simulink model "PassVeh14DOF"  (R2026b)
settings: Solver=ode23tb  StopTime=inf  FixedStep=.001  RelTol=1e-1  EnableMultiTasking=on
model workspace (MAT data in the model file):
  AlgnTrqCambCompl = [0 0 0 0]
  AlgnTrqSteerCompl = [0 0 0 0]
  AxlIxx = 62.3745166667
  AxlM = 160
  BumpCamber = [0 0 0 0]
  BumpCaster = [0 0 0 0]
  BumpSteer = [0 0 0 0]
  CambVsSteerAng = [0 0 0 0]
  CastVsSteerAng = [0 0 0 0]
  Cps = 2
  Cz = 5565.2246438
  CzWhlAxl = 11490.971257
  DCT_Param : object (value not decoded)
  Downshift_Speeds = [9.5625 12.9375 16.3125 19.6875 23.0625 26.4375 29.8125 33.1875 36.5625 39.9375 43.3125 46.6875 ... (28 elements, 4x7)]
  F0z = [2886 2907]
  F0zWhlAxl = 2907
  Hmax = 0.25
  Kz = 52451.0065793
  KzWhlAxl = 138031.612078
  LatCambCompl = [0 0 0 0]
  LatSteerCompl = [0 0 0 0]
  LatWhlCtrComplLat = [0 0 0 0]
  LatWhlCtrComplLng = [0  0  0  0; 0  0  0  0]
  LatWhlCtrDisp = [0 0 0 0]
  LngCambCompl = [0  0  0  0; 0  0  0  0]
  LngCastCompl = [0  0  0  0; 0  0  0  0]
  LngSteerCompl = [0  0  0  0; 0  0  0  0]
  LngWhlCtrCompl = [0  0  0  0; 0  0  0  0]
  LngWhlCtrDisp = [0 0 0 0]
  MotRatios = [1 1]
  NCyl = 6
  NrmlWhlFrcOff = [2886 2886 2907 2907]
  NrmlWhlRates = [52.4510065793 52.4510065793 52.4510065793 52.4510065793]
  Pedal_Positions = [0.1 0.4 0.5 0.9]
  Pstd = 101325
  Rair = 287
  RollCamber : object (value not decoded)
  RollCaster : object (value not decoded)
  RollSteer : object (value not decoded)
  RollStiffArb = [0 0]
  RollStiffArbFrnt = 800
  RollStiffNoArb = [0 0]
  RollStiffNoArbFrnt = 0
  RollStiffNoTwstRear = 0
  ShckFrcVsCompRate = [5.5652246438 5.5652246438 5.5652246438 5.5652246438]
  StatCamber = [0 0 0 0]
  StatCaster = [0 0 0 0]
  StatLdWhlR = [0.3 0.3 0.3 0.3]
  StatToe = [0 0 0 0]
  Trans : object (value not decoded)
  Tstd = 293.15
  Upshift_Speeds = [12.9375 16.3125 19.6875 33 26.4375 29.8125 33.1875 52.5 39.9375 43.3125 46.6875 77.25 ... (28 elements, 4x7)]
  VEH : object (value not decoded)
  Vd = 0.00346
  VrtLdTrnsfr = [0 0 0 0]
  WH : Mass (value not decoded)
  dt3D = 0.05
  f_air = [0 0 0 0 0 0 0 0 0 0 0 0 ... (256 elements, 16x16)]
  f_co = [0 0 0 0 0 0 0 0 0 0 0 0 ... (256 elements, 16x16)]
  f_co2 = [0 0 0 0 0 0 0 0 0 0 0 0 ... (256 elements, 16x16)]
  f_eff = [352.135682859 352.135682859 320.724378192 303.655312657 295.930136708 291.240087194 291.240271258 291.240312459 291.240275452 291.240198499 291.240100781 291.240018769 ... (256 elements, 16x16)]
  f_fuel = [0 0 0 0 0 0 0 0 0 0 0 0 ... (256 elements, 16x16)]
  f_hc = [0 0 0 0 0 0 0 0 0 0 0 0 ... (256 elements, 16x16)]
  f_nox = [0 0 0 0 0 0 0 0 0 0 0 0 ... (256 elements, 16x16)]
  f_pm = [0 0 0 0 0 0 0 0 0 0 0 0 ... (256 elements, 16x16)]
  f_susp_axl_bp = [1 2]
  f_susp_dz_bp = [-0.325022776267 -0.315022776267 -0.305022776267 -0.205022776267 -0.105022776267 -0.00502277626717 0.0949772237328 0.194977223733 0.204977223733 0.214977223733]
  f_susp_dzdot_bp = [-3 -0.3 -0.2 -0.1 0 0.1 0.2 0.3 3]
  f_susp_fmz = [-144070.391448 -93629.24037 -75929.1118915 -20630.5828179 -15385.48216 -10140.3815021 -4895.28084414 349.819813785 -31916.3973792 18437.6709544 -83996.1993354 -33555.0482577 ... (43920 elements, 10x9x61x2x4)]
  f_susp_geom = [0 0 0 0 0 0 0 0 0 0 0 0 ... (3660 elements, 10x61x2x3)]
  f_susp_strgdelta_bp = [-0.523598775598 -0.506145483078 -0.488692190558 -0.471238898038 -0.453785605519 -0.436332312999 -0.418879020479 -0.401425727959 -0.383972435439 -0.366519142919 -0.349065850399 -0.331612557879 ... (61 elements, 1x61)]
  f_tbrake = [0 76.8593923996 105.140482948 131.533638111 157.926793274 176.658631717 176.65727296 176.656856686 176.656879077 176.657093756 176.657404516 176.65772406 ... (256 elements, 16x16)]
  f_tbrake_n_bpt = [0 649.519052838 912.419621844 1175.32019085 1438.22075986 1701.12132886 1964.02189787 2226.92246687 2489.82303588 2752.72360489 3015.62417389 3278.5247429 ... (16 elements, 1x16)]
  f_tbrake_t_bpt = [0 34.6410161514 61.0341713143 87.4273264773 113.82048164 140.213636803 166.606791966 192.999947129 219.393102292 245.786257455 272.179412618 298.572567781 ... (16 elements, 1x16)]
  f_texh = [766.752464599 766.752464599 786.17542386 801.679939032 884.591982581 910.574397722 910.571871054 910.570774534 910.570601632 910.570821151 910.571247242 910.571639815 ... (256 elements, 16x16)]
  f_twc_eff_co = [0.17 0.25 0.45 0.99 0.99 0.99 0.99]
  f_twc_eff_hc = [0.21 0.375 0.75 0.98 0.98 0.98 0.98]
  f_twc_eff_lam = [0.909090909 0.944055944 0.979020979 1 1.013986014 1.048951049 1.083916084]
  f_twc_eff_nox = [0.98 0.98 0.98 0.97 0.05 0.02 0]
  numWheel = 4
symbols that are objects in the model workspace (value not decoded): VEH
libraries: vehdynlibtire x12, vehdynlibsuspension x8, autolibutils x5, sharedtransform x5, shared6dof x2, vehdynlibeom x1, vehdynlibtirecommon x1, matrix_library x1
(part 9 of 9)

== system PassVeh14DOF/Wheels and Tires/VDBS/Tires/MF Tires/Fz ==
  In1 : Inport
  In2 : Inport  Port=2
  In3 : Inport  Port=3
  In4 : Inport  Port=4
  Bus Selector{,1..3} (4 alike) : BusSelector  OutputSignals=Fz
  Vector Concatenate : Concatenate  NumInputs=4
  Out1 : Outport  VectorParamsAs1DForOutWhenUnconnected=off
  wires:
  Vector Concatenate/1 -> Out1/1
  In1/1 -> Bus Selector/1
  Bus Selector/1 -> Vector Concatenate/1  "<Fz>"
  In2/1 -> Bus Selector1/1
  In3/1 -> Bus Selector2/1
  In4/1 -> Bus Selector3/1
  Bus Selector1/1 -> Vector Concatenate/2  "<Fz>"
  Bus Selector2/1 -> Vector Concatenate/3  "<Fz>"
  Bus Selector3/1 -> Vector Concatenate/4  "<Fz>"

== system PassVeh14DOF/Wheels and Tires/VDBS/Tires/MF Tires/Mx ==
  In1 : Inport
  In2 : Inport  Port=2
  In3 : Inport  Port=3
  In4 : Inport  Port=4
  Bus Selector{,1..3} (4 alike) : BusSelector  OutputSignals=Mx
  Vector Concatenate : Concatenate  NumInputs=4
  Out1 : Outport  VectorParamsAs1DForOutWhenUnconnected=off
  wires:
  Vector Concatenate/1 -> Out1/1
  In1/1 -> Bus Selector/1
  Bus Selector/1 -> Vector Concatenate/1  "<Mx>"
  In2/1 -> Bus Selector1/1
  In3/1 -> Bus Selector2/1
  In4/1 -> Bus Selector3/1
  Bus Selector1/1 -> Vector Concatenate/2  "<Mx>"
  Bus Selector2/1 -> Vector Concatenate/3  "<Mx>"
  Bus Selector3/1 -> Vector Concatenate/4  "<Mx>"

== system PassVeh14DOF/Wheels and Tires/VDBS/Tires/MF Tires/My ==
  In1 : Inport
  In2 : Inport  Port=2
  In3 : Inport  Port=3
  In4 : Inport  Port=4
  Bus Selector{,1..3} (4 alike) : BusSelector  OutputSignals=My
  Vector Concatenate : Concatenate  NumInputs=4
  Out1 : Outport  VectorParamsAs1DForOutWhenUnconnected=off
  wires:
  Bus Selector3/1 -> Vector Concatenate/4  "<My>"
  Bus Selector2/1 -> Vector Concatenate/3  "<My>"
  Bus Selector1/1 -> Vector Concatenate/2  "<My>"
  In4/1 -> Bus Selector3/1
  In3/1 -> Bus Selector2/1
  In2/1 -> Bus Selector1/1
  Bus Selector/1 -> Vector Concatenate/1  "<My>"
  In1/1 -> Bus Selector/1
  Vector Concatenate/1 -> Out1/1

== system PassVeh14DOF/Wheels and Tires/VDBS/Tires/MF Tires/Mz ==
  In1 : Inport
  In2 : Inport  Port=2
  In3 : Inport  Port=3
  In4 : Inport  Port=4
  Bus Selector{,1..3} (4 alike) : BusSelector  OutputSignals=Mz
  Vector Concatenate : Concatenate  NumInputs=4
  Out1 : Outport  VectorParamsAs1DForOutWhenUnconnected=off
  wires:
  Bus Selector3/1 -> Vector Concatenate/4  "<Mz>"
  Bus Selector2/1 -> Vector Concatenate/3  "<Mz>"
  Bus Selector1/1 -> Vector Concatenate/2  "<Mz>"
  In4/1 -> Bus Selector3/1
  In3/1 -> Bus Selector2/1
  In2/1 -> Bus Selector1/1
  Bus Selector/1 -> Vector Concatenate/1  "<Mz>"
  In1/1 -> Bus Selector/1
  Vector Concatenate/1 -> Out1/1

== system PassVeh14DOF/Wheels and Tires/VDBS/Tires/MF Tires/Re ==
  In1 : Inport
  In2 : Inport  Port=2
  In3 : Inport  Port=3
  In4 : Inport  Port=4
  Bus Selector{,1..3} (4 alike) : BusSelector  OutputSignals=Re
  Vector Concatenate : Concatenate  NumInputs=4
  Out1 : Outport  VectorParamsAs1DForOutWhenUnconnected=off
  wires:
  Vector Concatenate/1 -> Out1/1
  In1/1 -> Bus Selector/1
  Bus Selector/1 -> Vector Concatenate/1  "<Re>"
  In2/1 -> Bus Selector1/1
  In3/1 -> Bus Selector2/1
  In4/1 -> Bus Selector3/1
  Bus Selector1/1 -> Vector Concatenate/2  "<Re>"
  Bus Selector2/1 -> Vector Concatenate/3  "<Re>"
  Bus Selector3/1 -> Vector Concatenate/4  "<Re>"

== system PassVeh14DOF/Wheels and Tires/VDBS/Tires/MF Tires/alpha ==
  In1 : Inport
  In2 : Inport  Port=2
  In3 : Inport  Port=3
  In4 : Inport  Port=4
  Bus Selector{,1..3} (4 alike) : BusSelector  OutputSignals=Alpha
  Vector Concatenate : Concatenate  NumInputs=4
  Out1 : Outport  VectorParamsAs1DForOutWhenUnconnected=off
  wires:
  Vector Concatenate/1 -> Out1/1
  In1/1 -> Bus Selector/1
  Bus Selector/1 -> Vector Concatenate/1  "<Alpha>"
  In2/1 -> Bus Selector1/1
  In3/1 -> Bus Selector2/1
  In4/1 -> Bus Selector3/1
  Bus Selector1/1 -> Vector Concatenate/2  "<Alpha>"
  Bus Selector2/1 -> Vector Concatenate/3  "<Alpha>"
  Bus Selector3/1 -> Vector Concatenate/4  "<Alpha>"

== system PassVeh14DOF/Wheels and Tires/VDBS/Tires/MF Tires/kappa ==
  In1 : Inport
  In2 : Inport  Port=2
  In3 : Inport  Port=3
  In4 : Inport  Port=4
  Bus Selector{,1..3} (4 alike) : BusSelector  OutputSignals=Kappa
  Vector Concatenate : Concatenate  NumInputs=4
  Out1 : Outport  VectorParamsAs1DForOutWhenUnconnected=off
  wires:
  Bus Selector3/1 -> Vector Concatenate/4  "<Kappa>"
  Bus Selector2/1 -> Vector Concatenate/3  "<Kappa>"
  Bus Selector1/1 -> Vector Concatenate/2  "<Kappa>"
  In4/1 -> Bus Selector3/1
  In3/1 -> Bus Selector2/1
  In2/1 -> Bus Selector1/1
  Bus Selector/1 -> Vector Concatenate/1  "<Kappa>"
  In1/1 -> Bus Selector/1
  Vector Concatenate/1 -> Out1/1

== system PassVeh14DOF/Wheels and Tires/VDBS/Tires/MF Tires/omega ==
  In1 : Inport
  In2 : Inport  Port=2
  In3 : Inport  Port=3
  In4 : Inport  Port=4
  Bus Selector{,1..3} (4 alike) : BusSelector  OutputSignals=Omega
  Vector Concatenate : Concatenate  NumInputs=4
  Out1 : Outport  VectorParamsAs1DForOutWhenUnconnected=off
  wires:
  In1/1 -> Bus Selector/1
  Bus Selector/1 -> Vector Concatenate/1  "<Omega>"
  In2/1 -> Bus Selector1/1
  In3/1 -> Bus Selector2/1
  In4/1 -> Bus Selector3/1
  Bus Selector1/1 -> Vector Concatenate/2  "<Omega>"
  Bus Selector2/1 -> Vector Concatenate/3  "<Omega>"
  Bus Selector3/1 -> Vector Concatenate/4  "<Omega>"
  Vector Concatenate/1 -> Out1/1

== system PassVeh14DOF/Wheels and Tires/VDBS/Tires/MF Tires/z ==
  In1 : Inport
  In2 : Inport  Port=2
  In3 : Inport  Port=3
  In4 : Inport  Port=4
  Bus Selector{,1..3} (4 alike) : BusSelector  OutputSignals=z
  Vector Concatenate : Concatenate  NumInputs=4
  Out1 : Outport  VectorParamsAs1DForOutWhenUnconnected=off
  wires:
  Bus Selector3/1 -> Vector Concatenate/4  "<z>"
  Bus Selector2/1 -> Vector Concatenate/3  "<z>"
  Bus Selector1/1 -> Vector Concatenate/2  "<z>"
  In4/1 -> Bus Selector3/1
  In3/1 -> Bus Selector2/1
  In2/1 -> Bus Selector1/1
  Bus Selector/1 -> Vector Concatenate/1  "<z>"
  In1/1 -> Bus Selector/1
  Vector Concatenate/1 -> Out1/1

== system PassVeh14DOF/Wheels and Tires/VDBS/Tires/MF Tires/zdot ==
  In1 : Inport
  In2 : Inport  Port=2
  In3 : Inport  Port=3
  In4 : Inport  Port=4
  Bus Selector{,1..3} (4 alike) : BusSelector  OutputSignals=zdot
  Vector Concatenate : Concatenate  NumInputs=4
  Out1 : Outport  VectorParamsAs1DForOutWhenUnconnected=off
  wires:
  Vector Concatenate/1 -> Out1/1
  In1/1 -> Bus Selector/1
  Bus Selector/1 -> Vector Concatenate/1  "<zdot>"
  In2/1 -> Bus Selector1/1
  In3/1 -> Bus Selector2/1
  In4/1 -> Bus Selector3/1
  Bus Selector1/1 -> Vector Concatenate/2  "<zdot>"
  Bus Selector2/1 -> Vector Concatenate/3  "<zdot>"
  Bus Selector3/1 -> Vector Concatenate/4  "<zdot>"

== matlab function PassVeh14DOF/Vehicle/Suspension to Chasiss Transforms/Estimated Unsprung Mass Orientation ==
  data: angles output size=3; angleIn input size=3; GeomXYZ output size=3; GemoXYZIn input size=3; Ground input size=4; trackW parameter; wheelB parameter
function [angles,GeomXYZ]= three26(angleIn, GemoXYZIn, Ground,trackW, wheelB)%#codegen
coder.allowpcode('plain')
% Copyright 2018 The MathWorks, Inc.
[angles,GeomXYZ]= vdynthree2six(angleIn, GemoXYZIn, Ground,trackW, wheelB);

== matlab function PassVeh14DOF/Wheels and Tires/VDBS/Veh2Tire/Camber Angle ==
  data: u input; y output
function y = fcn(u)
temp = squeeze(u(3,2:3,:));
y=atan(temp(1,:)./temp(2,:))';
